simulink model "sf_resolve_signal_object"  (R2025b)
settings: Solver=FixedStepDiscrete  StartTime=0.0  StopTime=5  FixedStep=1  RelTol=1e-3  EnableMultiTasking=on
PostLoadFcn:
  | load sf_resolve_signal_object_data;
settings Model: ExtModeAutoUpdateStatusClock=off  Creator=The MathWorks, Inc.  LastModifiedBy=The MathWorks, Inc.
settings SolverCC: AlgebraicLoopSolver=TrustRegion
settings DataIOCC: LimitDataPoints=on  SaveFormat=Array  ReturnWorkspaceOutputs=off
settings OptimizationCC: ReuseModelBlockBuffer=off  ExpressionDepthLimit=2147483647.0  InitFltsAndDblsToZero=on  EfficientMapNaN2IntZero=off  LifeSpan=inf
settings DebuggingCC: UnderspecifiedInitializationDetection=Classic  MergeDetectMultiDrivingBlocksExec=none  FcnCallInpInsideContextMsg=warning  UnconnectedInputMsg=warning  UnconnectedOutputMsg=warning  UnconnectedLineMsg=warning  StateNameClashWarn=warning  SFUnexpectedBacktrackingDiag=warning  SFNoUnconditionalDefaultTransitionDiag=warning  SFExecutionAtInitializationDiag=none  ArithmeticOperatorsInVariantConditions=warning
settings HardwareCC: ProdBitPerPointer=32.0  ProdBitPerSizeT=32.0  ProdBitPerPtrDiffT=32.0  ProdLargestAtomicFloat=None  ProdIntDivRoundTo=Undefined  ProdEndianess=Unspecified  ProdWordSize=32.0  ProdHWDeviceType=32-bit Generic
settings ModelReferenceCC: EnableRefExpFcnMdlSchedulingChecks=on  PropagateSignalLabelsOutOfModel=off
settings SFSimCC: SimUseLocalCustomCode=off  SimParseCustomCode=off  CustomCodeUndefinedFunction=UseInterfaceOnly
settings RTWCC: GenerateReport=on  RTWUseLocalCustomCode=off  LaunchReport=on  GPUComputeCapability=3.5  DLArmComputeVersion=19.05
settings CodeAppCC: StateflowObjectComments=on
settings GRTTargetCC: TargetLangStandard=C89/C90 (ANSI)  CombineOutputUpdateFcns=off  GRTInterface=on
settings ConfigComp: CovMetricSettings=dw  CovSaveCumulativeToWorkspaceVar=on  CovSaveSingleToWorkspaceVar=on  CovExternalEMLEnable=off  CovSFcnEnable=off

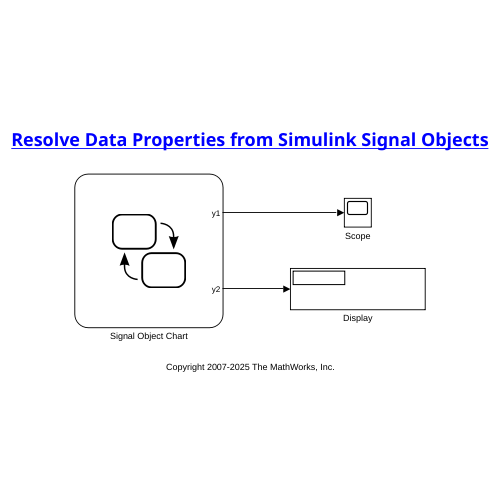
[thumbnail: Simulink's stored preview of the top-level diagram]
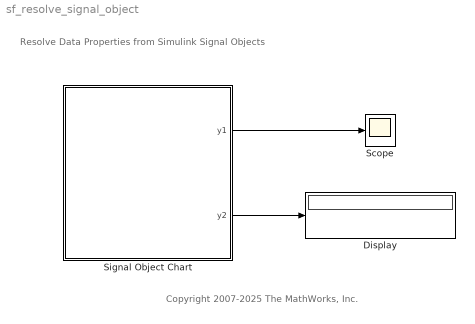
== system sf_resolve_signal_object ==
  note: Copyright 2007-2025 The MathWorks, Inc.
  note: Resolve Data Properties from Simulink Signal Objects
  Display : Display
  Scope : Scope
      settings: ActiveDisplayYMinimum=15  ActiveDisplayYMaximum=17
  Signal Object Chart : Stateflow chart  TreatAsAtomicUnit=on
  wires:
  Signal Object Chart/1(y1) -> Scope/1
  Signal Object Chart/2(y2) -> Display/1

== stateflow chart sf_resolve_signal_object/Signal Object Chart ==
  state S
    en: y1 = 2 * (local + 10);
    du: y2 = 5;
  (default) -> S
  data: local local double; y1 output double; y2 output double
